simulink model "Boost_Thevenin_Equivalent"  (R2024b)
settings: Solver=FixedStepAuto  StartTime=0.0  StopTime=4  MaxStep=1e-4  RelTol=1e-3
libraries: spsCurrentMeasurementLib x3, spsSeriesRLCBranchLib x3, spsVoltageMeasurementLib x3, slpidlib x2, spsPWMGeneratorDCDCLib x2, spsDCVoltageSourceLib x1, spsDiodeLib x1, spsMosfetLib x1, spspowerguiLib x1
settings Model: Creator=Parti  LastModifiedBy=Eng.Abd-Elrhman Saad

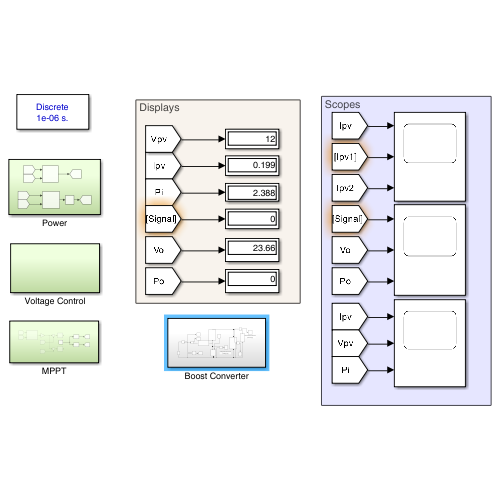
[thumbnail: Simulink's stored preview of the top-level diagram]
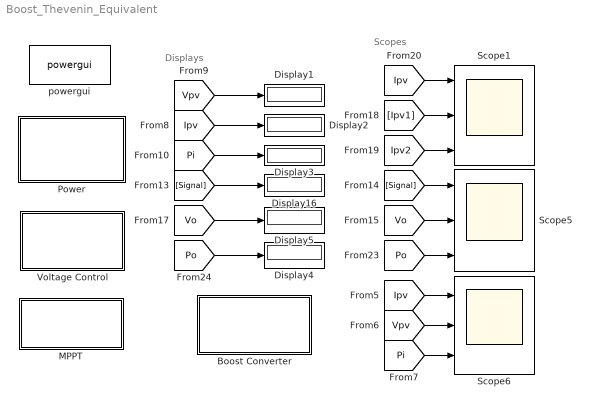
== system Boost_Thevenin_Equivalent ==
  note: Scopes
  note: Displays
  Boost Converter : Subsystem
  Display{1..5,16} (6 alike) : Display
  MPPT : Subsystem
  Power : Subsystem
  Scope1 : Scope  NumInputPorts=3
  Scope5 : Scope  NumInputPorts=3
  Scope6 : Scope  NumInputPorts=3
  Voltage Control : Subsystem
  powergui : spspowerguiLib/powergui  Priority=1  SimulationMode=Discrete  SampleTime=1e-6  frequency=60  Iterations=50  frequencyindice=0  Pbase=100e6  ErrMax=1e-4  UnitsV=kV  UnitsW=MW  buscounter=0  FunctionMessages=off  echomessages=off  EnableUseOfTLC=off  CurrentSourceSwitches=off  DisableSnubberDevices=off  DisableRonSwitches=off  DisableVfSwitches=off  DisplayEquations=off  AutomaticDiscreteSolvers=off  SolverType=Tustin/Backward Euler (TBE)  Interpol=off  ExternalGateDelay=off  methode=off  Ts=100  x0status=blocks  SPID=on  SwTol=0  HookPort=off  NonlinearTolerance=1e-4  nMaxIteration=100  ContinueOnMaxIteration=off  RestoreLinks=warning  ResistiveCurrentMeasurement=off  Frange=[0:2:500]  Ylog=off  Xlog=on  ShowGrid=off  save=off  variable=ZData  structure=0  ZoomFFT=off  StartTime=0.0  cycles=1  DisplayStyle=1  fundamental=60  FreqAxis=off  MaxFrequency=1000  frequencyindicesteady=1  RmsSteady=1  display=off
  wires:
  [Vpv] -> Scope6/2
  [Pi] -> Scope6/3
  [Ipv] -> Scope6/1
  [Ipv] -> Display2/1
  [Vpv] -> Display1/1
  [Pi] -> Display3/1
  [Signal] -> Display16/1
  [Signal] -> Scope5/1
  [Ipv1] -> Scope1/2
  [Ipv] -> Scope1/1
  [Ipv2] -> Scope1/3
  [Vo] -> Scope5/2
  [Vo] -> Display5/1
  [Po] -> Scope5/3
  [Po] -> Display4/1

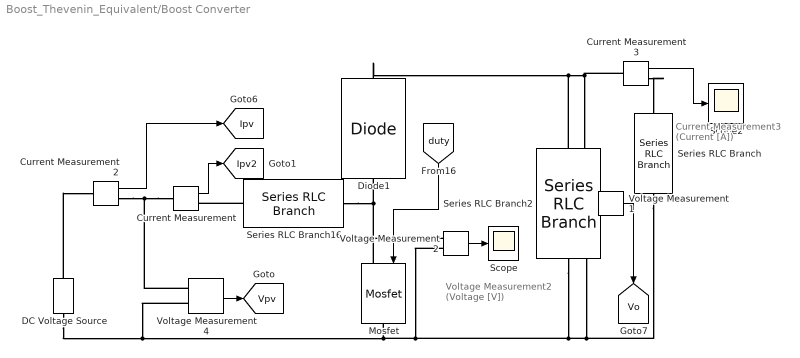
== system Boost_Thevenin_Equivalent/Boost Converter ==
  note: Voltage Measurement2
      | (Voltage [V])
  note: Current Measurement3
      | (Current [A])
  Current Measurement : spsCurrentMeasurementLib/Current Measurement  PhasorSimulation=off  OutputType=Complex  PSBequivalent=0
  Current Measurement2 : spsCurrentMeasurementLib/Current Measurement  PhasorSimulation=off  OutputType=Complex  PSBequivalent=0
  Current Measurement3 : spsCurrentMeasurementLib/Current Measurement  PhasorSimulation=off  OutputType=Complex  PSBequivalent=0
  DC Voltage Source : spsDCVoltageSourceLib/DC Voltage Source  Amplitude=12  Measurements=None
  Diode1 : spsDiodeLib/Diode  Ron=0.001  Lon=0  Vf=0.8  IC=0  UseSnubber=0  Rs=500  Cs=250e-9  Measurements=off
  Mosfet : spsMosfetLib/Mosfet  Ron=0.1  Lon=0  Rd=0.01  Vfd=0  IC=0  Rs=1e5  Cs=inf  Measurements=off
  Scope : Scope
  Scope2 : Scope
  Series RLC Branch : spsSeriesRLCBranchLib/Series RLC Branch  LConnTagsString=__new0  RConnTagsString=__new0  BranchType=R  Resistance=220  Inductance=1e-3  SetiL0=off  InitialCurrent=0  Capacitance=1e-6  Setx0=off  InitialVoltage=0  Measurements=None
  Series RLC Branch16 : spsSeriesRLCBranchLib/Series RLC Branch  LConnTagsString=__new0  RConnTagsString=__new0  BranchType=L  Resistance=1  Inductance=2e-3  SetiL0=off  InitialCurrent=0  Capacitance=1000e-6  Setx0=on  InitialVoltage=100  Measurements=None
  Series RLC Branch2 : spsSeriesRLCBranchLib/Series RLC Branch  LConnTagsString=__new0  RConnTagsString=__new0  BranchType=C  Resistance=1  Inductance=1e-3  SetiL0=off  InitialCurrent=0  Capacitance=2e-3  Setx0=on  InitialVoltage=0  Measurements=None
  Voltage Measurement1 : spsVoltageMeasurementLib/Voltage Measurement  PhasorSimulation=off  OutputType=Complex  PSBequivalent=0
  Voltage Measurement2 : spsVoltageMeasurementLib/Voltage Measurement  PhasorSimulation=off  OutputType=Complex  PSBequivalent=0
  Voltage Measurement4 : spsVoltageMeasurementLib/Voltage Measurement  PhasorSimulation=off  OutputType=Complex  PSBequivalent=0
  tag scope: Ipv2=global, Ipv=global, Vo=global, Vpv=global
  wires:
  Voltage Measurement4/1 -> [Vpv]
  Voltage Measurement1/1 -> [Vo]
  Voltage Measurement2/1 -> Scope/1
  Current Measurement3/1 -> Scope2/1
  Current Measurement/1 -> [Ipv2]
  [duty] -> Mosfet/1
  Current Measurement2/1 -> [Ipv]
  connections:
  Current Measurement3/RConn1 -- Series RLC Branch/LConn1
  Series RLC Branch16/RConn1 -- Mosfet/LConn1 -- Voltage Measurement2/LConn1 -- Diode1/LConn1
  Series RLC Branch2/RConn1 -- Voltage Measurement2/LConn2 -- DC Voltage Source/LConn1 -- Voltage Measurement4/LConn2 -- Mosfet/RConn1 -- Series RLC Branch/RConn1 -- Voltage Measurement1/LConn2
  Diode1/RConn1 -- Series RLC Branch2/LConn1 -- Voltage Measurement1/LConn1 -- Current Measurement3/LConn1
  Current Measurement/LConn1 -- Current Measurement2/RConn1 -- Voltage Measurement4/LConn1
  DC Voltage Source/RConn1 -- Current Measurement2/LConn1
  Series RLC Branch16/LConn1 -- Current Measurement/RConn1

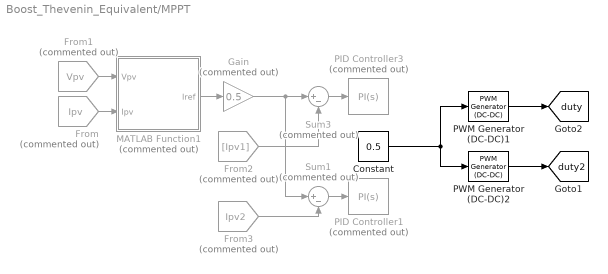
== system Boost_Thevenin_Equivalent/MPPT ==
  Constant : Constant  Value=0.5
  From : From  Commented=on  GotoTag=Ipv  TagVisibility=global
  From1 : From  Commented=on  GotoTag=Vpv  TagVisibility=global
  From2 : From  Commented=on  GotoTag=Ipv1  TagVisibility=global
  From3 : From  Commented=on  GotoTag=Ipv2  TagVisibility=global
  Gain : Gain  Commented=on  Gain=0.5
  MATLAB Function1 : MATLAB Function  Commented=on  TreatAsAtomicUnit=on
  PID Controller1 : slpidlib/PID Controller  Commented=on  Controller=PI  Form=Parallel  TimeDomain=Continuous-time  UseExternalTs=off  SampleTime=-1  IntegratorMethod=Forward Euler  FilterMethod=Forward Euler  ControllerParametersSource=internal  P=-0.1  I=-1  UseKiTs=off  D=0  UseExternalDerivativeSource=off  N=100  UseFilter=on  TunerSelectOption=Transfer Function Based (PID Tuner App)  InitialConditionSource=internal  InitialConditionForIntegrator=0  InitialConditionForFilter=0  DifferentiatorICPrevScaledInput=0  ExternalReset=none  TrackingMode=off  Kt=1  LimitOutput=off  SatLimitsSource=internal  UpperSaturationLimit=1  LowerSaturationLimit=0  LinearizeAsGain=on  AntiWindupMode=clamping  Kb=1  LimitIntegrator=off  UpperIntegratorSaturationLimit=inf  LowerIntegratorSaturationLimit=-inf  POutMin=[]  POutMax=[]  IOutMin=[]  IOutMax=[]  DOutMin=[]  DOutMax=[]  NOutMin=[]  NOutMax=[]  SumOutMin=[]  SumOutMax=[]  SaturationOutMin=[]  SaturationOutMax=[]  PParamMin=[]  PParamMax=[]  IParamMin=[]  IParamMax=[]  DParamMin=[]  DParamMax=[]  NParamMin=[]  NParamMax=[]  KbParamMin=[]  KbParamMax=[]  KtParamMin=[]  KtParamMax=[]  KbOutMin=[]  KbOutMax=[]  KtOutMin=[]  KtOutMax=[]  IntegratorOutMin=[]  IntegratorOutMax=[]  FilterOutMin=[]  FilterOutMax=[]  SumI1OutMin=[]  SumI1OutMax=[]  SumI2OutMin=[]  SumI2OutMax=[]  SumI3OutMin=[]  SumI3OutMax=[]  SumI4OutMin=[]  SumI4OutMax=[]  SumDOutMin=[]  SumDOutMax=[]  DifferentiatorOutMin=[]  DifferentiatorOutMax=[]  FilterDiffOutCoefMin=[]  FilterDiffOutCoefMax=[]  ReciprocalOutMin=[]  ReciprocalOutMax=[]  SumDenOutMin=[]  SumDenOutMax=[]  SumNumOutMin=[]  SumNumOutMax=[]  DivideOutMin=[]  DivideOutMax=[]  UdiffTsProdOutMin=[]  UdiffTsProdOutMax=[]  NTsProdOutMin=[]  NTsProdOutMax=[]  UintegralTsProdOutMin=[]  UintegralTsProdOutMax=[]  UngainTsProdOutMin=[]  UngainTsProdOutMax=[]  ClampingZeroOutDataTypeStr=Inherit: Inherit via back propagation  ClampingZeroOutMin=[]  ClampingZeroOutMax=[]  FilterDenConstantOutDataTypeStr=Inherit: Inherit via back propagation  FilterDenConstantOutMin=[]  FilterDenConstantOutMax=[]  PCopyOutDataTypeStr=Inherit: Inherit via back propagation  PCopyOutMin=[]  PCopyOutMax=[]  NCopyOutDataTypeStr=Inherit: Inherit via back propagation  NCopyOutMin=[]  NCopyOutMax=[]  IntegratorContinuousStateAttributes=''  IntegratorStateMustResolveToSignalObject=off  IntegratorRTWStateStorageClass=Auto  FilterContinuousStateAttributes=''  FilterStateMustResolveToSignalObject=off  FilterRTWStateStorageClass=Auto  ParallelPVariant=InternalParameters  IdealPVariant=Disabled  IVariant=InternalParameters  DVariant=Disabled  IntegratorVariant=Continuous  SatVariant=Disabled  AWVariant=Passthrough  PCopyVariant=Disabled  TRVariant=Disabled  FdbkBlocksVariant=Forward  IdealPFdbkVariant=Disabled  SatFdbkVariant=Disabled  DerivativeFilterVariant=Disabled  NVariant=Disabled  NCopyVariant=Disabled_SignalSpec  FilterICVariant=Disabled  IntegratorICVariant=InternalICs  ExternalResetVariant=Disabled  TRSumVariant=Passthrough  SumFdbkVariant=Disabled  SumVariant=Sum_PI  TsampFilterVariant=InternalTs  TsampNgainVariant=Passthrough  TsampIntegralVariant=Disabled_SignalSpec  ExternalSaturationOutDataTypeStr=Inherit: Same as second input  DerivativeSourceVariant=Disabled  PreIntVariant=InternalPreInt
  PID Controller3 : slpidlib/PID Controller  Commented=on  Controller=PI  Form=Parallel  TimeDomain=Continuous-time  UseExternalTs=off  SampleTime=-1  IntegratorMethod=Forward Euler  FilterMethod=Forward Euler  ControllerParametersSource=internal  P=1  I=10  UseKiTs=off  D=0  UseExternalDerivativeSource=off  N=100  UseFilter=on  TunerSelectOption=Transfer Function Based (PID Tuner App)  InitialConditionSource=internal  InitialConditionForIntegrator=0  InitialConditionForFilter=0  DifferentiatorICPrevScaledInput=0  ExternalReset=none  TrackingMode=off  Kt=1  LimitOutput=off  SatLimitsSource=internal  UpperSaturationLimit=1  LowerSaturationLimit=0  LinearizeAsGain=on  AntiWindupMode=clamping  Kb=1  LimitIntegrator=off  UpperIntegratorSaturationLimit=inf  LowerIntegratorSaturationLimit=-inf  POutMin=[]  POutMax=[]  IOutMin=[]  IOutMax=[]  DOutMin=[]  DOutMax=[]  NOutMin=[]  NOutMax=[]  SumOutMin=[]  SumOutMax=[]  SaturationOutMin=[]  SaturationOutMax=[]  PParamMin=[]  PParamMax=[]  IParamMin=[]  IParamMax=[]  DParamMin=[]  DParamMax=[]  NParamMin=[]  NParamMax=[]  KbParamMin=[]  KbParamMax=[]  KtParamMin=[]  KtParamMax=[]  KbOutMin=[]  KbOutMax=[]  KtOutMin=[]  KtOutMax=[]  IntegratorOutMin=[]  IntegratorOutMax=[]  FilterOutMin=[]  FilterOutMax=[]  SumI1OutMin=[]  SumI1OutMax=[]  SumI2OutMin=[]  SumI2OutMax=[]  SumI3OutMin=[]  SumI3OutMax=[]  SumI4OutMin=[]  SumI4OutMax=[]  SumDOutMin=[]  SumDOutMax=[]  DifferentiatorOutMin=[]  DifferentiatorOutMax=[]  FilterDiffOutCoefMin=[]  FilterDiffOutCoefMax=[]  ReciprocalOutMin=[]  ReciprocalOutMax=[]  SumDenOutMin=[]  SumDenOutMax=[]  SumNumOutMin=[]  SumNumOutMax=[]  DivideOutMin=[]  DivideOutMax=[]  UdiffTsProdOutMin=[]  UdiffTsProdOutMax=[]  NTsProdOutMin=[]  NTsProdOutMax=[]  UintegralTsProdOutMin=[]  UintegralTsProdOutMax=[]  UngainTsProdOutMin=[]  UngainTsProdOutMax=[]  ClampingZeroOutDataTypeStr=Inherit: Inherit via back propagation  ClampingZeroOutMin=[]  ClampingZeroOutMax=[]  FilterDenConstantOutDataTypeStr=Inherit: Inherit via back propagation  FilterDenConstantOutMin=[]  FilterDenConstantOutMax=[]  PCopyOutDataTypeStr=Inherit: Inherit via back propagation  PCopyOutMin=[]  PCopyOutMax=[]  NCopyOutDataTypeStr=Inherit: Inherit via back propagation  NCopyOutMin=[]  NCopyOutMax=[]  IntegratorContinuousStateAttributes=''  IntegratorStateMustResolveToSignalObject=off  IntegratorRTWStateStorageClass=Auto  FilterContinuousStateAttributes=''  FilterStateMustResolveToSignalObject=off  FilterRTWStateStorageClass=Auto  ParallelPVariant=InternalParameters  IdealPVariant=Disabled  IVariant=InternalParameters  DVariant=Disabled  IntegratorVariant=Continuous  SatVariant=Disabled  AWVariant=Passthrough  PCopyVariant=Disabled  TRVariant=Disabled  FdbkBlocksVariant=Forward  IdealPFdbkVariant=Disabled  SatFdbkVariant=Disabled  DerivativeFilterVariant=Disabled  NVariant=Disabled  NCopyVariant=Disabled_SignalSpec  FilterICVariant=Disabled  IntegratorICVariant=InternalICs  ExternalResetVariant=Disabled  TRSumVariant=Passthrough  SumFdbkVariant=Disabled  SumVariant=Sum_PI  TsampFilterVariant=InternalTs  TsampNgainVariant=Passthrough  TsampIntegralVariant=Disabled_SignalSpec  ExternalSaturationOutDataTypeStr=Inherit: Same as second input  DerivativeSourceVariant=Disabled  PreIntVariant=InternalPreInt
  PWM Generator (DC-DC)1 : spsPWMGeneratorDCDCLib/PWM Generator (DC-DC)  Fsw=30000  Ts=1e-6
  PWM Generator (DC-DC)2 : spsPWMGeneratorDCDCLib/PWM Generator (DC-DC)  Fsw=30000  Ts=1e-6
  Sum1 : Sum  Commented=on  Inputs=|+-
  Sum3 : Sum  Commented=on  Inputs=|+-
  tag scope: duty2=global, duty=global
  wires:
  From1/1 -> MATLAB Function1/1(Vpv)
  PWM Generator (DC-DC)1/1 -> [duty]
  MATLAB Function1/1(Iref) -> Gain/1
  From/1 -> MATLAB Function1/2(Ipv)
  Sum3/1 -> PID Controller3/1
  From2/1 -> Sum3/2
  From3/1 -> Sum1/2
  Gain/1 -> Sum1/1, Sum3/1
  Sum1/1 -> PID Controller1/1
  PWM Generator (DC-DC)2/1 -> [duty2]
  Constant/1 -> PWM Generator (DC-DC)1/1, PWM Generator (DC-DC)2/1

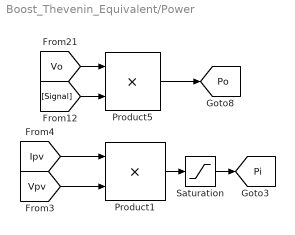
== system Boost_Thevenin_Equivalent/Power ==
  Product1 : Product
  Product5 : Product
  Saturation : Saturate  UpperLimit=199.85  LowerLimit=0
  tag scope: Pi=global, Po=global
  wires:
  Saturation/1 -> [Pi]
  [Ipv] -> Product1/1
  [Signal] -> Product5/2
  [Vo] -> Product5/1
  Product1/1 -> Saturation/1
  Product5/1 -> [Po]
  [Vpv] -> Product1/2

== system Boost_Thevenin_Equivalent/Voltage Control ==

== matlab function Boost_Thevenin_Equivalent/MPPT/MATLAB Function1 ==
  data: Vpv input; Ipv input; Iref output
function Iref = mppt(Vpv, Ipv)
    persistent V_target Pmax Vbest mode timer;
    
    Ts = 1e-6;
    
    % Finer voltage sweep for better resolution
    V_oc_est = 21.5;
    V_scan_min = 17.4;
    V_ramp_rate = 150;          
    
    if isempty(V_target)
        V_target = V_oc_est;
        Pmax = 0;
        Vbest = 17.5;
        mode = 0;
        timer = 0;
    end
    
    Ppv = Vpv * Ipv;
    
    switch mode
        case 0
            V_target = V_oc_est;
            Pmax = 0;
            if Vpv > 21       % Relaxed threshold
                mode = 1;
            end
            
        case 1
            % Record power with interpolation for better peak detection
            if Ppv > Pmax
                Pmax = Ppv;
                Vbest = V_target;
            end
            
            V_target = V_target - (V_ramp_rate * Ts);
            
            if V_target <= V_scan_min
                mode = 2;
            end
            
        case 2
            if V_target < Vbest
                V_target = V_target + (100 * Ts);  % Slower, more accurate return
            else
                V_target = Vbest;
                mode = 3;
                timer = 0;
            end
            
        case 3
            timer = timer + Ts;
            if timer >= 5.0
                mode = 0;
            end
    end
    
    persistent err_int;
    if isempty(err_int), err_int = 0; end
    
    err = Vpv - V_target;
    err_int = err_int + err * Ts;
    err_int = max(min(err_int, 15), -15);
    
    % Higher proportional gain to reduce steady-state error
    Kp = 0.5;        % Increased from 0.1 for better tracking
    Ki = 150;        % Slightly reduced to prevent oscillation
    
    % Adjusted base current closer to expected MPP
    I_calc = 3 + Kp * err + Ki * err_int;
    
    Iref = max(min(I_calc, 12.18), 0);
end
